simulink model "stabilizer_bar_repair"  (R2023a)
settings: Solver=ode4  StartTime=0  StopTime=40  FixedStep=Ts_plant  MaxStep=0.001  RelTol=1e-3
InitFcn:
  | run(fullfile(fileparts(get_param(bdroot,'FileName')),'a001_new_Design_LQR_Controller.m'));
values from neighbouring files (symbols this model uses):
  cycle_cfg = jsondecode(fileread(fullfile(repair_root,'repair_support','repair_cycle_bank.json')))    [a001_new_Design_LQR_Controller.m]
  entry_cfg = rmfield(entry_bank_source,{'labels','source_hashes','note','source_par_sha256'})    [a001_new_Design_LQR_Controller.m]
  path_geometry = repair_build_geometry(path_cfg)    [a001_new_Design_LQR_Controller.m]
  path_Q = diag([10,10,2])    [a001_new_Design_LQR_Controller.m]
  path_R = diag([100,100,10])    [a001_new_Design_LQR_Controller.m]
  repair_cfg = struct    [a001_new_Design_LQR_Controller.m]
  repair_simfile = 'C:\Users\Public\Documents\CarSim2020.0_Data\Extensions\Simulink\00carsim_workspace\009\stabilizer_bar\simfile.sim'    [a001_new_Design_LQR_Controller.m]
  stadium_cfg = jsondecode(fileread(fullfile(repair_root,'repair_support','repair_stadium_reference.json')))    [a001_new_Design_LQR_Controller.m]
  Ts = 0.01    [a001_new_Design_LQR_Controller.m]
  Ts_plant = 0.0005    [a001_new_Design_LQR_Controller.m]
undefined symbols (not defined in the file or in its folder): path_cfg
(part 1 of 2)
settings Model: Creator=28583  LastModifiedBy=28583

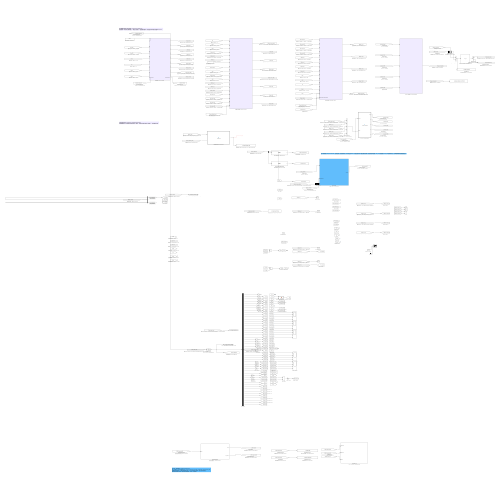
[thumbnail: Simulink's stored preview of the top-level diagram]
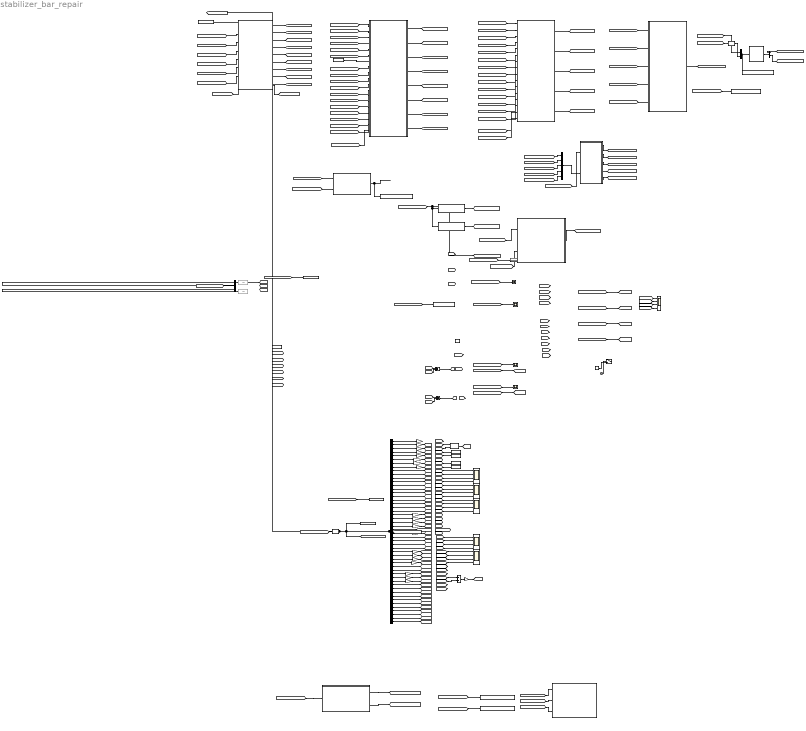
== system stabilizer_bar_repair ==
  note: 第四章路径跟踪与分阶段维修 / Chapter 4 Staged Repair
      | 路径跟踪 → 状态与力需求修正 → 轮速/力矩执行 → 直接前轮角接口。跨层信号均采用本层局部Goto/From。
  note: 诊断与实际状态 / Diagnostics and Measured States
      | 保留原始需求、修正残差和未滤波数据；无候选、轮荷失效或坐标失效立即停止，不开展增益扫描。
  note: 起漂与局部维持 / Entry & Local Hold：工程试验支路，路径反馈关闭。工作点来自当前CarSim；先建立后轴滑移，再建立横摆与负侧偏，最后按实测状态接管。drift_entry仅起漂维持；drift_cycle按实测状态门控，经卸载和解除转弯后接管普通直行。
  note: 第一阶段：固定软硬组合 / Fixed Active Roll Study
      | 唯一入口a001；asb_case选择baseline、front_soft_rear_hard、soft_soft、hard_hard、front_hard_rear_soft。
      | 原漂移控制与路线冻结，新增支路按0.0005s执行。CarSim内部384/384不动，输出比较不预设优劣。
      | 跨区信号均为本层local标签；新增支路不增加滤波、延迟或人为表端停止。
  ASBExportSplit : Demux  Outputs=[50 26]
      settings: AttributesFormatString=原50路与新增26路 / Split Export
  ASBImport12 : Mux  Inputs=2
      settings: AttributesFormatString=12路CarSim输入 / Import Twelve
  ASBImportOrder : Selector  InputPortWidth=4  IndexOptions=Index vector (dialog)  Indices=[1 3 2 4]  OutputSizes=1
      settings: AttributesFormatString=GUI轮序重排 / GUI Force Order
  ActiveRollMonitor : Subsystem
      settings: AttributesFormatString=主动稳定杆诊断面板 / Active Roll Monitor
  ActiveRollResearch : Subsystem
      settings: AttributesFormatString=理想主动稳定杆 / Ideal Active Roll
  ActualStateSample 车辆状态采样模块 : ZeroOrderHold  SampleTime=Ts
      settings: AttributesFormatString=|
      | ActualStateSample
      | 车辆状态采样模块 / ActualStateSample
  Add : Sum
      settings: AttributesFormatString=Add / Add
  Add1 : Sum
      settings: AttributesFormatString=Add1 / Add1
  Add2 : Sum
      settings: AttributesFormatString=Add2 / Add2
  CarSim S-Function : S-Function  Priority=1  FunctionName=vs_sf  Parameters=repair_simfile,2,0  SFunctionDeploymentMode=off  EnableBusSupport=off
      settings: AttributesFormatString=CarSim S-Function / CarSimSFunction
  CarSimInterface : Subsystem
      settings: AttributesFormatString=CarSim八路接口 / CarSimInterface
  Clock : Clock
      settings: AttributesFormatString=Clock / Clock
  Constant1 : Constant  Value=Ts
      settings: AttributesFormatString=Constant1 / Constant1
  Constant8 : Constant  Value=-7.37
      settings: AttributesFormatString=Constant8 / Constant8
  Demux : Demux  Outputs=50
      settings: AttributesFormatString=Demux / Demux
  Display : Display
      settings: AttributesFormatString=Display / Display
  EntryLocalMode : Subsystem
      settings: AttributesFormatString=起漂维持退出与直行 / Drift Cycle
  EntryModeSelector : MATLAB Function  TreatAsAtomicUnit=on
      settings: AttributesFormatString=运行模式选择 / Mode Selection
  Gain1 : Gain  Gain=1/3.6
      settings: AttributesFormatString=Gain1 / Gain1
  Gain{7,10..12,16,18..20} (8 alike) : Gain  Gain=pi/30
      Gain10 settings: AttributesFormatString=Gain10 / Gain10
      Gain11 settings: AttributesFormatString=Gain11 / Gain11
      Gain12 settings: AttributesFormatString=Gain12 / Gain12
      Gain16 settings: AttributesFormatString=Gain16 / Gain16
      Gain18 settings: AttributesFormatString=Gain18 / Gain18
      Gain19 settings: AttributesFormatString=Gain19 / Gain19
      Gain20 settings: AttributesFormatString=Gain20 / Gain20
      Gain7 settings: AttributesFormatString=Gain7 / Gain7
  Gain{4..6,9,13,21..22} (7 alike) : Gain  Gain=pi/180
      Gain13 settings: AttributesFormatString=Gain13 / Gain13
      Gain21 settings: AttributesFormatString=Gain21 / Gain21
      Gain22 settings: AttributesFormatString=Gain22 / Gain22
      Gain4 settings: AttributesFormatString=Gain4 / Gain4
      Gain5 settings: AttributesFormatString=Gain5 / Gain5
      Gain6 settings: AttributesFormatString=Gain6 / Gain6
      Gain9 settings: AttributesFormatString=Gain9 / Gain9
  Gain14 : Gain  Gain=1/3.6
      settings: AttributesFormatString=Gain14 / Gain14
  Gain15 : Gain  Gain=9.80665
      settings: AttributesFormatString=Gain15 / Gain15
  Gain2 : Gain  Gain=1/3.6
      settings: AttributesFormatString=Gain2 / Gain2
  Gain3 : Gain  Gain=9.80665
      settings: AttributesFormatString=Gain3 / Gain3
  Gain8 : Gain  Gain=1/2
      settings: AttributesFormatString=Gain8 / Gain8
  LegacyCommand5 : Mux  Inputs=5
      settings: AttributesFormatString=原模式指令 / Legacy Commands
  LogASBDiagnostics : ToWorkspace  VariableName=asb_diag  SaveFormat=Structure With Time  SampleTime=-1
      settings: AttributesFormatString=记录力矩功率残差 / Log ASB Diagnostics
  LogASBImport : ToWorkspace  VariableName=asb_import12  SaveFormat=Structure With Time  SampleTime=-1
      settings: AttributesFormatString=记录12路实际输入 / Log Full Import
  LogASBSuspension : ToWorkspace  VariableName=asb_suspension  SaveFormat=Structure With Time  SampleTime=-1
      settings: AttributesFormatString=记录悬架26路 / Log Suspension
  Log_repair_actuator_command : ToWorkspace  VariableName=repair_actuator_command  SaveFormat=Timeseries  SampleTime=-1
      settings: AttributesFormatString=Log_repair_actuator_command / Log_repair_actuator_command
  Log_repair_path_diag : ToWorkspace  VariableName=repair_path_diag  SaveFormat=Timeseries  SampleTime=-1
      settings: AttributesFormatString=原始路径日志 / Log_repair_path_diag
  Log_repair_plant_raw : ToWorkspace  VariableName=repair_plant_raw  SaveFormat=Timeseries  SampleTime=-1
      settings: AttributesFormatString=Log_repair_plant_raw / Log_repair_plant_raw
  Log_repair_plant_sampled : ToWorkspace  VariableName=repair_plant_sampled  SaveFormat=Timeseries  SampleTime=-1
      settings: AttributesFormatString=Log_repair_plant_sampled / Log_repair_plant_sampled
  Log_repair_reference_log : ToWorkspace  VariableName=repair_reference_log  SaveFormat=Timeseries  SampleTime=-1
      settings: AttributesFormatString=Log_repair_reference_log / Log_repair_reference_log
  Log_repair_stage_stop : ToWorkspace  VariableName=repair_stage_stop  SaveFormat=Timeseries  SampleTime=-1
      settings: AttributesFormatString=原始记录 repair_stage_stop / Log_repair_stage_stop
  MATLAB Function : MATLAB Function  TreatAsAtomicUnit=on
      settings: AttributesFormatString=MATLAB Function / MATLABFunction
  MeasuredFourWheelLoads : Selector  InputPortWidth=50  IndexOptions=Index vector (dialog)  Indices=17:20  OutputSizes=1
      settings: AttributesFormatString=四轮实际轮荷 / Measured Fz [N]
  PathClock : DigitalClock  SampleTime=Ts
      settings: AttributesFormatString=控制采样时刻 / PathClock
  ReferenceSignals : Demux  Outputs=3
      settings: AttributesFormatString=ReferenceSignals / ReferenceSignals
  RepairClock : DigitalClock  SampleTime=Ts
      settings: AttributesFormatString=控制采样时刻 / RepairClock
  RepairTs : Constant  Value=Ts
      settings: AttributesFormatString=控制周期参数 / RepairTs
  Scope{,2,7,9,13,21} (6 alike) : Scope  NumInputPorts=4
      Scope settings: AttributesFormatString=Scope / Scope
      Scope13 settings: AttributesFormatString=Scope13 / Scope13
      Scope2 settings: AttributesFormatString=Scope2 / Scope2
      Scope21 settings: AttributesFormatString=Scope21 / Scope21
      Scope7 settings: AttributesFormatString=Scope7 / Scope7
      Scope9 settings: AttributesFormatString=Scope9 / Scope9
  Scope{14..17} (4 alike) : Scope
      Scope14 settings: AttributesFormatString=Scope14 / Scope14
      Scope15 settings: AttributesFormatString=Scope15 / Scope15
      Scope16 settings: AttributesFormatString=Scope16 / Scope16
      Scope17 settings: AttributesFormatString=Scope17 / Scope17
  StageStop : MATLAB Function  Description=|  TreatAsAtomicUnit=on
      | 停止逻辑已移除 / Stop logic removed
      | 阶段状态仅作为日志信号，CarSim/求解器按自身行为终止。
      settings: AttributesFormatString=分阶段停止条件 / StageStop
  Switch : Switch  Criteria=u2 > Threshold  Threshold=0.5  SaturateOnIntegerOverflow=off  InputSameDT=off
      settings: AttributesFormatString=Switch / Switch
  To Workspace1 : ToWorkspace  VariableName=beta_out1  SaveFormat=Timeseries  SampleTime=-1
      settings: AttributesFormatString=To Workspace1 / ToWorkspace1
  To Workspace2 : ToWorkspace  VariableName=AVz_out1  SaveFormat=Timeseries  SampleTime=-1
      settings: AttributesFormatString=To Workspace2 / ToWorkspace2
  To Workspace3 : ToWorkspace  VariableName=Roll_out1  SaveFormat=Timeseries  SampleTime=-1
      settings: AttributesFormatString=To Workspace3 / ToWorkspace3
  To Workspace4 : ToWorkspace  VariableName=Ay_out1  SaveFormat=Timeseries  SampleTime=-1
      settings: AttributesFormatString=To Workspace4 / ToWorkspace4
  Transfer Fcn1 : TransferFcn  Commented=through  Denominator=[1 1]
  Transfer Fcn2 : TransferFcn  Commented=through  Denominator=[1 1]
  WheelContactSelector : Selector  InputPortWidth=50  IndexOptions=Index vector (dialog)  Indices=[9 10 11 12 17 18 19 20]  OutputSizes=1
      settings: AttributesFormatString=轮胎负载与轮荷 / Wheel Contact
  执行器调节层 : Subsystem  Description=|
      | 执行命令直通 / Unbounded Commands to CarSim
      | 关闭外加转角、角速度、轮速变化及轮端力矩限幅。
      | 非有限值和CarSim求解器错误由CarSim/求解器本身反映。
      settings: AttributesFormatString=执行器调节 / Actuator Control
  路径跟踪层 : Subsystem  Description=|
      | 普通工况mode=6：直线→平滑左转→直线。
      | 漂移权重与侧偏参考始终为零。
      | 主链仍为参考对齐→位姿误差→LQR→期望状态；保留原控制增益。
      settings: AttributesFormatString=路径跟踪 / Path Tracking
  车辆运动控制层 : Subsystem  Description=|
      | 状态参考直通 / Unconstrained Reference Pass-through
      | 完整LQR状态命令不再经过33点可行域搜索、5%轴力残差门槛或摩擦圆投影。
      | CarSim实际Fx/Fy/Fz、滑移和车辆状态用于判断命令后果。
      settings: AttributesFormatString=车辆运动控制 / Motion Control
  wires:
  ActualStateSample 车辆状态采样模块/1 -> Demux/1, [Repair_sampled_plant], [Repair_HeldPlant], Log_repair_plant_sampled/1, [Stadium_Measured]
  Add/1 -> [Fzf]
  Add1/1 -> [Fzr]
  Add2/1 -> Gain8/1
  [Ay] -> To Workspace4/1
  CarSimInterface/1(CarSimInputs) -> [Repair_commands]
  Clock/1 -> Switch/2
  Constant8/1 -> Switch/3
  Demux/1 -> Gain14/1
  Demux/2 -> Gain1/1
  Demux/3 -> Gain2/1
  Demux/4 -> Gain4/1
  Demux/5 -> Gain5/1
  Demux/6 -> Gain3/1
  Demux/7 -> Gain15/1
  Demux/8 -> Gain6/1
  Demux/9 -> [Fx_L1]
  Demux/10 -> [Fx_R1]
  Demux/11 -> [Fx_L2]
  Demux/12 -> [Fx_R2]
  Demux/13 -> [Fy_L1]
  Demux/14 -> [Fy_R1]
  Demux/15 -> [Fy_L2]
  Demux/16 -> [Fy_R2]
  Demux/17 -> [Fz_L1]
  Demux/18 -> [Fz_R1]
  Demux/19 -> [Fz_L2]
  Demux/20 -> [Fz_R2]
  Demux/21 -> Gain16/1
  Demux/22 -> Gain18/1
  Demux/23 -> Gain19/1
  Demux/24 -> Gain20/1
  Demux/25 -> [Steer_wheel_angular_rate]
  Demux/26 -> Gain9/1
  Demux/27 -> [Kappa_L1]
  Demux/28 -> [Kappa_R1]
  Demux/29 -> [Kappa_L2]
  Demux/30 -> [Kappa_R2]
  Demux/31 -> Gain7/1
  Demux/32 -> Gain10/1
  Demux/33 -> Gain11/1
  Demux/34 -> Gain12/1
  Demux/35 -> [Xcg_TM]
  Demux/36 -> [Ycg_TM]
  Demux/37 -> Gain13/1
  Demux/38 -> Gain21/1
  Demux/39 -> Gain22/1
  Demux/40 -> [Xo]
  Demux/41 -> [Yo]
  Demux/42 -> [My_Dr_L1]
  Demux/43 -> [My_Dr_R1]
  Demux/44 -> [My_Dr_L2]
  Demux/45 -> [My_Dr_R2]
  Demux/46 -> [Alpha_L1]
  Demux/47 -> [Alpha_R1]
  Demux/48 -> [Alpha_L2]
  Demux/49 -> [Alpha_R2]
  Demux/50 -> [Steer_SW]
  [wheel_steer_L1] -> Add2/1
  [Fz_L1] -> Add/1
  [Fz_R1] -> Add/2
  [Fz_L2] -> Add1/1
  [Fz_R2] -> Add1/2
  [wheel_steer_R1] -> Add2/2
  [IMP_MY_OUT_L1] -> Scope7/1
  [IMP_MY_OUT_R1] -> Scope7/2
  [AVy_wheel_L1] -> Scope21/1
  [IMP_MY_OUT_L2] -> Scope7/3
  [IMP_MY_OUT_R2] -> Scope7/4
  [AVy_wheel_R1] -> Scope21/2
  [AVy_wheel_L2] -> Scope21/3
  [AVy_wheel_R2] -> Scope21/4
  [Fx_L1] -> Scope9/1
  [Fx_L2] -> Scope9/3
  [Fx_R1] -> Scope9/2
  [Fx_R2] -> Scope9/4
  [Fy_L1] -> Scope2/1
  [Fy_L2] -> Scope2/3
  [Fy_R1] -> Scope2/2
  [Fy_R2] -> Scope2/4
  [Fz_L1] -> Scope/1
  [Fz_L2] -> Scope/3
  [Fz_R1] -> Scope/2
  [Fz_R2] -> Scope/4
  Gain1/1 -> [Vx]
  Gain10/1 -> [AVy_wheel_R1]
  Gain11/1 -> [AVy_wheel_L2]
  Gain12/1 -> [AVy_wheel_R2]
  Gain13/1 -> [Yaw]
  Gain15/1 -> [Ay]
  Gain16/1 -> [AVy_L1]
  Gain18/1 -> [AVy_R1]
  Gain19/1 -> [AVy_L2]
  Gain2/1 -> [Vy]
  Gain20/1 -> [AVy_R2]
  Gain21/1 -> [wheel_steer_L1]
  Gain22/1 -> [wheel_steer_R1]
  Gain3/1 -> [Ax]
  Gain4/1 -> [beta]
  Gain5/1 -> [AVz]
  Gain6/1 -> [Roll]
  Gain7/1 -> [AVy_wheel_L1]
  Gain8/1 -> [delta_acutal_F]
  Gain9/1 -> [AVx]
  [Kappa_L1] -> Scope13/1
  [Kappa_L2] -> Scope13/3
  [Kappa_R1] -> Scope13/2
  [Kappa_R2] -> Scope13/4
  MATLAB Function/1(V) -> [V]
  [Repair_plant_raw] -> ActualStateSample 车辆状态采样模块/1
  [Repair_inverse_status] -> Display/1
  [Repair_T_FL] -> [IMP_MY_OUT_L1]
  [Repair_T_FR] -> [IMP_MY_OUT_R1]
  [Repair_T_RL] -> [IMP_MY_OUT_L2]
  [Repair_Fxf] -> [Fxf_desire]
  [Repair_Fxr] -> [Fxr_desire]
  [Repair_T_RR] -> [IMP_MY_OUT_R2]
  [Repair_plant_raw] -> Log_repair_plant_raw/1
  [Repair_path_diag] -> Log_repair_path_diag/1
  [Repair_nominal] -> Log_repair_reference_log/1
  [Repair_nominal] -> ReferenceSignals/1
  [Repair_commands] -> Log_repair_actuator_command/1
  [Repair_sampled_plant] -> StageStop/2(plant)
  [Repair_wf] -> Scope14/1
  [Repair_wr] -> Scope15/1
  [Repair_Fxf] -> Scope16/1
  [Repair_Fxr] -> Scope17/1
  [Repair_valid] -> StageStop/1(valid)
  [Fzr] -> 执行器调节层/10(后轴垂向力)
  [Repair_blend] -> 车辆运动控制层/10(漂移模式1_0drift_mode)
  [Fzf] -> 车辆运动控制层/11(前轴垂向载荷Fzf)
  [V] -> 执行器调节层/11(V)
  [Repair_ey] -> 车辆运动控制层/12(PathLateralError)
  [beta] -> 执行器调节层/12(beta)
  [AVz] -> 执行器调节层/13(r)
  [Repair_chi] -> 车辆运动控制层/13(PathCourseError)
  [Repair_alpha] -> 执行器调节层/14(期望前轮侧偏角alpha_f_d)
  [Repair_kappa] -> 车辆运动控制层/14(PathCurvature)
  [AVy_wheel_L1] -> 车辆运动控制层/15(WheelSpeed1)
  [AVy_wheel_R1] -> 车辆运动控制层/16(WheelSpeed2)
  [AVy_wheel_L2] -> 车辆运动控制层/17(WheelSpeed3)
  [AVy_wheel_R2] -> 车辆运动控制层/18(WheelSpeed4)
  [AVy_wheel_L1] -> 执行器调节层/1(左前轮实际轮速)
  [V] -> 车辆运动控制层/1(实际速度V)
  [AVy_wheel_R1] -> 执行器调节层/2(右前轮实际轮速)
  [Xcg_TM] -> 路径跟踪层/2(Xcg)
  [beta] -> 车辆运动控制层/2(质心侧偏角beta)
  [AVy_wheel_L2] -> 执行器调节层/3(左后轮实际轮速)
  [AVz] -> 车辆运动控制层/3(横摆角速度r)
  [Ycg_TM] -> 路径跟踪层/3(Ycg)
  [AVy_wheel_R2] -> 执行器调节层/4(右后轮实际轮速)
  [Repair_Vxd] -> 车辆运动控制层/4(路径跟踪层输出的期望纵向速度Vxd)
  [Yaw] -> 路径跟踪层/4(Yaw)
  [Repair_Vyd] -> 车辆运动控制层/5(路径跟踪层输出的期望侧向速度Vyd)
  [Repair_wf] -> 执行器调节层/5(前轴期望轴轮速)
  [V] -> 路径跟踪层/5(Speed)
  [Repair_rd] -> 车辆运动控制层/6(路径跟踪层输出的期望横摆角速度rd_in)
  [Repair_wr] -> 执行器调节层/6(后轴期望轴轮速)
  [beta] -> 路径跟踪层/6(Beta)
  [AVz] -> 路径跟踪层/7(YawRate)
  [Repair_Fxf] -> 执行器调节层/7(前轴期望纵向力)
  [Repair_Fxr] -> 执行器调节层/8(后轴期望纵向力)
  [delta_acutal_F] -> 车辆运动控制层/8(前轮转角delta_f)
  [Fzf] -> 执行器调节层/9(前轴垂向力)
  [Fzr] -> 车辆运动控制层/9(后轴垂向载荷Fzr)
  ReferenceSignals/1 -> [V_refer]
  ReferenceSignals/2 -> Transfer Fcn1/1
  ReferenceSignals/3 -> Transfer Fcn2/1
  RepairClock/1 -> 路径跟踪层/1(Time)
  RepairTs/1 -> 车辆运动控制层/7(采样时间)
  [Roll] -> To Workspace3/1
  StageStop/1(stop) -> Log_repair_stage_stop/1
  [Vx] -> MATLAB Function/1(Vx)
  [Vy] -> MATLAB Function/2(Vy)
  [beta] -> To Workspace1/1
  [AVz] -> To Workspace2/1
  执行器调节层/1(左前轮驱动力矩) -> [Repair_T_FL]
  执行器调节层/2(右前轮驱动力矩) -> [Repair_T_FR]
  执行器调节层/3(左后轮驱动力矩) -> [Repair_T_RL]
  执行器调节层/4(右后轮驱动力矩) -> [Repair_T_RR]
  执行器调节层/5(FrontAngleCommand) -> [Repair_delta_target]
  路径跟踪层/1(Vxd) -> [Repair_Vxd]
  路径跟踪层/2(Vyd) -> [Repair_Vyd]
  路径跟踪层/3(rd) -> [Repair_rd]
  路径跟踪层/4(LateralError) -> [Repair_ey]
  路径跟踪层/5(CourseError) -> [Repair_chi]
  路径跟踪层/6(ProjectedCurvature) -> [Repair_kappa]
  路径跟踪层/7(DriftBlend) -> [Repair_blend]
  路径跟踪层/8(PathDiagnostics) -> [Repair_path_diag]
  路径跟踪层/9(NominalStates) -> [Repair_nominal]
  车辆运动控制层/1(漂移状态status) -> [Repair_inverse_status]
  车辆运动控制层/2(期望前轴轮速1) -> [Repair_wf]
  车辆运动控制层/3(期望后轴轮速1) -> [Repair_wr]
  车辆运动控制层/4(期望前轮侧偏角2) -> [Repair_alpha]
  车辆运动控制层/5(轮胎反演状态1) -> [Repair_force_valid]
  车辆运动控制层/6(期望前轮纵向力Fxf) -> [Repair_Fxf]
  车辆运动控制层/7(期望后轮纵向力Fxr) -> [Repair_Fxr]
  车辆运动控制层/8(Feasible) -> [Repair_valid]
  WheelContactSelector/1 -> [Repair_WheelContact]
  [Repair_WheelContact] -> 车辆运动控制层/19(MeasuredWheelContact)
  [Repair_WheelContact] -> 执行器调节层/15(MeasuredWheelContact)
  [Repair_HeldPlant] -> WheelContactSelector/1, MeasuredFourWheelLoads/1, [entry_plant50]
  MeasuredFourWheelLoads/1 -> [measured_Fz4]
  [measured_Fz4] -> 执行器调节层/16(MeasuredFourWheelLoads)
  [Repair_delta_target] -> LegacyCommand5/1
  [Repair_T_FL] -> LegacyCommand5/2
  [Repair_T_FR] -> LegacyCommand5/3
  [Repair_T_RL] -> LegacyCommand5/4
  [Repair_T_RR] -> LegacyCommand5/5
  [entry_command5] -> EntryModeSelector/1(newcmd)
  LegacyCommand5/1 -> EntryModeSelector/2(oldcmd)
  EntryModeSelector/1(angle) -> [selected_Angle]
  [selected_Angle] -> CarSimInterface/1(Input1)
  EntryModeSelector/2(tfl) -> [selected_TFL]
  [selected_TFL] -> CarSimInterface/2(Input2)
  EntryModeSelector/3(tfr) -> [selected_TFR]
  [selected_TFR] -> CarSimInterface/3(Input3)
  EntryModeSelector/4(trl) -> [selected_TRL]
  [selected_TRL] -> CarSimInterface/4(Input4)
  EntryModeSelector/5(trr) -> [selected_TRR]
  [selected_TRR] -> CarSimInterface/5(Input5)
  [entry_plant50] -> EntryLocalMode/1(y)
  EntryLocalMode/1(command) -> [entry_command5]
  [Stadium_Measured] -> 路径跟踪层/8(StadiumRaw)
  路径跟踪层/10(StadiumPacket) -> [Stadium_Packet]
  [Stadium_Packet] -> EntryLocalMode/2(StadiumPacket)
  [Repair_commands] -> ASBImport12/1
  [ASB_Force4] -> ASBImportOrder/1
  ASBImportOrder/1 -> ASBImport12/2
  ASBImport12/1 -> CarSim S-Function/1, LogASBImport/1
  CarSim S-Function/1 -> ASBExportSplit/1
  ASBExportSplit/1 -> [Repair_plant_raw]
  ASBExportSplit/2 -> [ASB_Suspension26]
  [ASB_Suspension26] -> ActiveRollResearch/1(Raw)
  ActiveRollResearch/1(Forces) -> [ASB_Force4]
  ActiveRollResearch/2(Diagnostics) -> [ASB_Diagnostics44]
  [ASB_Diagnostics44] -> LogASBDiagnostics/1
  [ASB_Suspension26] -> LogASBSuspension/1
  [ASB_Diagnostics44] -> ActiveRollMonitor/1(Diagnostics)
  [ASB_Suspension26] -> ActiveRollMonitor/2(Suspension)
  [Repair_plant_raw] -> ActiveRollMonitor/3(Vehicle)

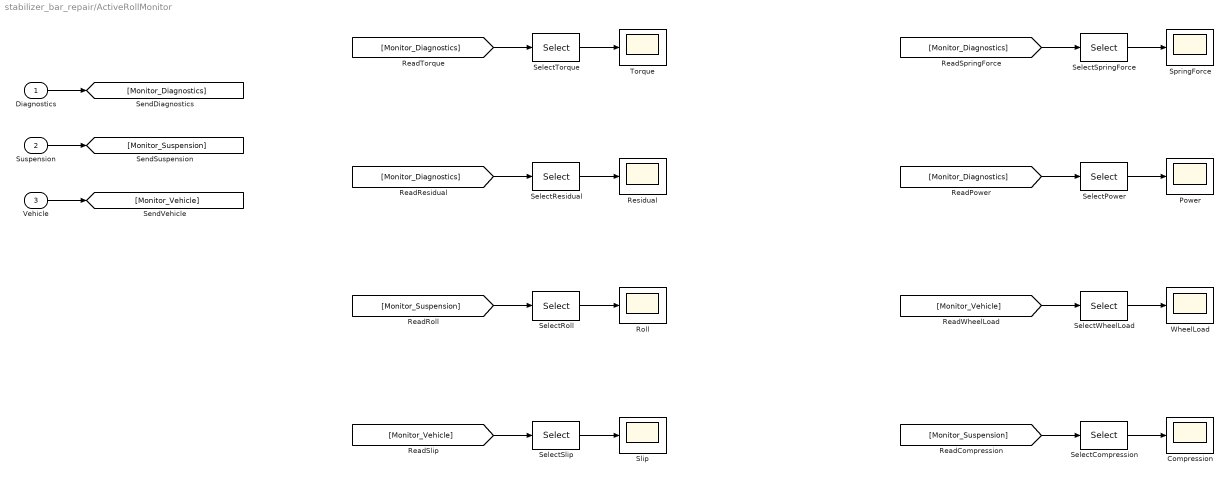
== system stabilizer_bar_repair/ActiveRollMonitor ==
  Diagnostics : Inport  PortDimensions=44
      settings: AttributesFormatString=44项物理诊断 / Diagnostics
  Suspension : Inport  Port=2  PortDimensions=26
      settings: AttributesFormatString=26路悬架测量 / Suspension
  Vehicle : Inport  Port=3  PortDimensions=50
      settings: AttributesFormatString=50路车辆测量 / Vehicle
  Compression : Scope
      settings: AttributesFormatString=|
      | 四轮弹簧压缩 mm
      | Spring Compression
  Power : Scope
      settings: AttributesFormatString=|
      | 两口径机械功率与差值 W
      | Power
  Residual : Scope
      settings: AttributesFormatString=|
      | 力矩残差Nm与合力N
      | Residual
  Roll : Scope
      settings: AttributesFormatString=|
      | 相对侧倾deg及速度deg每秒
      | Relative Roll
  SelectCompression : Selector  InputPortWidth=26  IndexOptions=Index vector (dialog)  Indices=[17:20]  OutputSizes=1
      settings: AttributesFormatString=选取 / Select
  SelectPower : Selector  InputPortWidth=44  IndexOptions=Index vector (dialog)  Indices=[29:34]  OutputSizes=1
      settings: AttributesFormatString=选取 / Select
  SelectResidual : Selector  InputPortWidth=44  IndexOptions=Index vector (dialog)  Indices=[11 12 27 28]  OutputSizes=1
      settings: AttributesFormatString=选取 / Select
  SelectRoll : Selector  InputPortWidth=26  IndexOptions=Index vector (dialog)  Indices=[1:4]  OutputSizes=1
      settings: AttributesFormatString=选取 / Select
  SelectSlip : Selector  InputPortWidth=50  IndexOptions=Index vector (dialog)  Indices=[27:30]  OutputSizes=1
      settings: AttributesFormatString=选取 / Select
  SelectSpringForce : Selector  InputPortWidth=44  IndexOptions=Index vector (dialog)  Indices=[19:26]  OutputSizes=1
      settings: AttributesFormatString=选取 / Select
  SelectTorque : Selector  InputPortWidth=44  IndexOptions=Index vector (dialog)  Indices=[7:10]  OutputSizes=1
      settings: AttributesFormatString=选取 / Select
  SelectWheelLoad : Selector  InputPortWidth=50  IndexOptions=Index vector (dialog)  Indices=[17:20]  OutputSizes=1
      settings: AttributesFormatString=选取 / Select
  Slip : Scope
      settings: AttributesFormatString=|
      | 四轮纵滑比
      | Longitudinal Slip
  SpringForce : Scope
      settings: AttributesFormatString=|
      | 四轮输入与实际弹簧力 N
      | Spring Force
  Torque : Scope
      settings: AttributesFormatString=|
      | 前后目标与实际力矩 Nm
      | Torque
  WheelLoad : Scope
      settings: AttributesFormatString=|
      | 四轮法向载荷 N
      | Wheel Load
  wires:
  Diagnostics/1 -> [Monitor_Diagnostics]
  Suspension/1 -> [Monitor_Suspension]
  Vehicle/1 -> [Monitor_Vehicle]
  [Monitor_Diagnostics] -> SelectTorque/1
  SelectTorque/1 -> Torque/1
  [Monitor_Diagnostics] -> SelectSpringForce/1
  SelectSpringForce/1 -> SpringForce/1
  [Monitor_Diagnostics] -> SelectResidual/1
  SelectResidual/1 -> Residual/1
  [Monitor_Diagnostics] -> SelectPower/1
  SelectPower/1 -> Power/1
  [Monitor_Suspension] -> SelectRoll/1
  SelectRoll/1 -> Roll/1
  [Monitor_Vehicle] -> SelectWheelLoad/1
  SelectWheelLoad/1 -> WheelLoad/1
  [Monitor_Vehicle] -> SelectSlip/1
  SelectSlip/1 -> Slip/1
  [Monitor_Suspension] -> SelectCompression/1
  SelectCompression/1 -> Compression/1

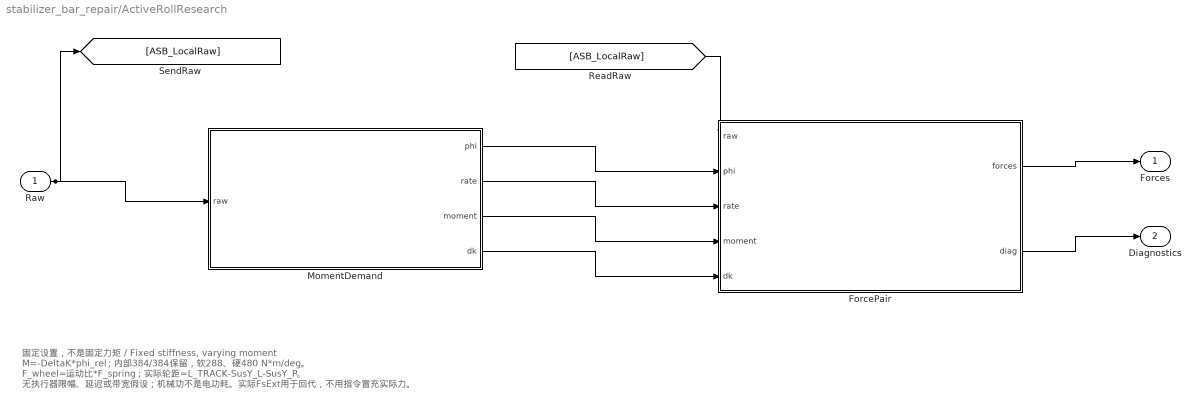
== system stabilizer_bar_repair/ActiveRollResearch ==
  note: 固定设置，不是固定力矩 / Fixed stiffness, varying moment
      | M=-DeltaK*phi_rel；内部384/384保留，软288、硬480 N*m/deg。
      | F_wheel=运动比*F_spring；实际轮距=L_TRACK-SusY_L-SusY_R。
      | 无执行器限幅、延迟或带宽假设；机械功不是电功耗。实际FsExt用于回代，不用指令冒充实际力。
  Raw : Inport  PortDimensions=26
      settings: AttributesFormatString=悬架26路 / Suspension Raw
  ForcePair : MATLAB Function  TreatAsAtomicUnit=on
      settings: AttributesFormatString=运动比力偶与回代 / Force Pair
  MomentDemand : MATLAB Function  TreatAsAtomicUnit=on
      settings: AttributesFormatString=固定刚度与恢复力矩 / Moment Demand
  Forces : Outport
      settings: AttributesFormatString=弹簧力FL FR RL RR / Spring Forces
  Diagnostics : Outport  Port=2
      settings: AttributesFormatString=44项物理诊断 / Diagnostics
  wires:
  Raw/1 -> MomentDemand/1(raw), [ASB_LocalRaw]
  [ASB_LocalRaw] -> ForcePair/1(raw)
  MomentDemand/1(phi) -> ForcePair/2(phi)
  MomentDemand/2(rate) -> ForcePair/3(rate)
  MomentDemand/3(moment) -> ForcePair/4(moment)
  MomentDemand/4(dk) -> ForcePair/5(dk)
  ForcePair/1(forces) -> Forces/1
  ForcePair/2(diag) -> Diagnostics/1

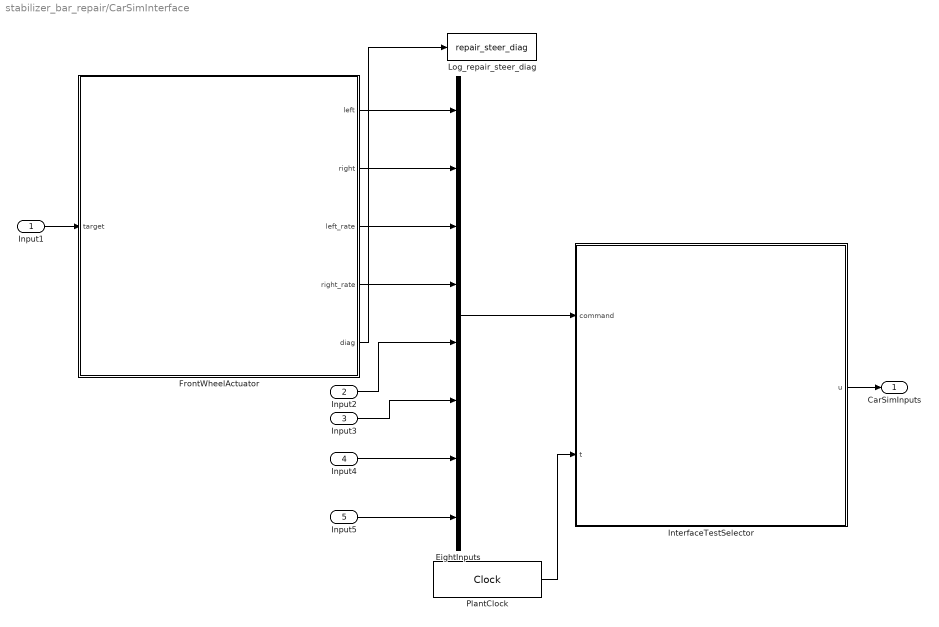
== system stabilizer_bar_repair/CarSimInterface ==
  Input1 : Inport
      settings: AttributesFormatString=Repair_delta_target / Input1
  Input2 : Inport  Port=2
      settings: AttributesFormatString=Repair_T_FL / Input2
  Input3 : Inport  Port=3
      settings: AttributesFormatString=Repair_T_FR / Input3
  Input4 : Inport  Port=4
      settings: AttributesFormatString=Repair_T_RL / Input4
  Input5 : Inport  Port=5
      settings: AttributesFormatString=Repair_T_RR / Input5
  EightInputs : Mux  Inputs=8
      settings: AttributesFormatString=CarSim输入顺序 / EightInputs
  FrontWheelActuator : MATLAB Function  TreatAsAtomicUnit=on
      settings: AttributesFormatString=前轮角与角速度 / FrontWheelActuator
  InterfaceTestSelector : MATLAB Function  TreatAsAtomicUnit=on
      settings: AttributesFormatString=显式接口短测选择 / InterfaceTestSelector
  Log_repair_steer_diag : ToWorkspace  VariableName=repair_steer_diag  SaveFormat=Timeseries  SampleTime=-1
      settings: AttributesFormatString=原始记录 repair_steer_diag / Log_repair_steer_diag
  PlantClock : DigitalClock  SampleTime=Ts_plant
      settings: AttributesFormatString=交换时刻 / PlantClock
  CarSimInputs : Outport
      settings: AttributesFormatString=八路导入向量 / CarSimInputs
  wires:
  Input3/1 -> EightInputs/6
  EightInputs/1 -> InterfaceTestSelector/1(command)
  Input2/1 -> EightInputs/5
  InterfaceTestSelector/1(u) -> CarSimInputs/1
  Input1/1 -> FrontWheelActuator/1(target)
  FrontWheelActuator/5(diag) -> Log_repair_steer_diag/1
  FrontWheelActuator/1(left) -> EightInputs/1
  FrontWheelActuator/2(right) -> EightInputs/2
  FrontWheelActuator/3(left_rate) -> EightInputs/3
  FrontWheelActuator/4(right_rate) -> EightInputs/4
  PlantClock/1 -> InterfaceTestSelector/2(t)
  Input4/1 -> EightInputs/7
  Input5/1 -> EightInputs/8

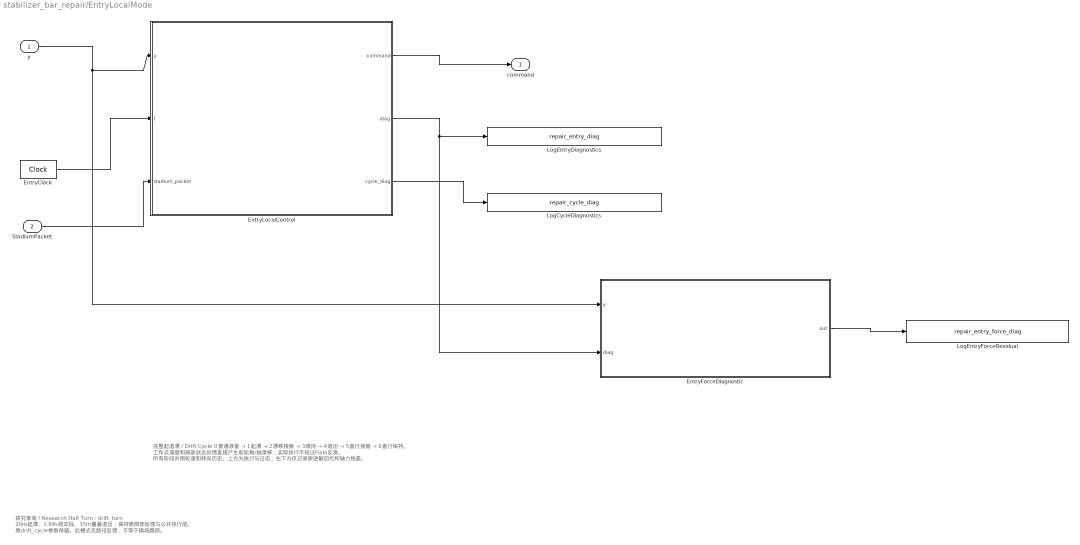
== system stabilizer_bar_repair/EntryLocalMode ==
  note: 完整起退漂 / Drift Cycle
      | 0普通准备 → 1起漂 → 2漂移接管 → 3维持 → 4退出 → 5直行接管 → 6直行保持。
      | 工作点调度和局部状态反馈直接产生前轮角/轴滑移；实际执行不经过Fiala反演。
      | 所有阶段共用轮速和转向历史。上方为执行与日志；右下方仅记录原逆解回代和轴力残差。
  note: 研究单弯 / Research Half Turn：drift_turn
      | 20m起漂、1.84s稳定段、35m重叠退出；保持原局部反馈与公共执行层。
      | 原drift_cycle参数保留。此模式无路径反馈，不等于操场跟踪。
  y : Inport
      settings: AttributesFormatString=实测状态 / Measured Plant
  StadiumPacket : Inport  Port=2
      settings: AttributesFormatString=操场执行参考 / Stadium Packet
  EntryClock : DigitalClock  SampleTime=Ts
      settings: AttributesFormatString=控制时钟 / Control Clock
  EntryForceDiagnostic : MATLAB Function  TreatAsAtomicUnit=on
      settings: AttributesFormatString=原逆解回代与力残差 / Inverse & Force Residual
  EntryLocalControl : MATLAB Function  TreatAsAtomicUnit=on
      settings: AttributesFormatString=五项状态反馈与执行 / Five-State Feedback and Execution
  LogCycleDiagnostics : ToWorkspace  VariableName=repair_cycle_diag  SaveFormat=Structure With Time  SampleTime=-1
      settings: AttributesFormatString=退出与直行接管记录 / Cycle Diagnostics
  LogEntryDiagnostics : ToWorkspace  VariableName=repair_entry_diag  SaveFormat=Structure With Time  SampleTime=-1
      settings: AttributesFormatString=起漂与接管记录 / Entry Diagnostics
  LogEntryForceResidual : ToWorkspace  VariableName=repair_entry_force_diag  SaveFormat=Structure With Time  SampleTime=-1
      settings: AttributesFormatString=轴力与回代记录 / Force Residual Log
  command : Outport
      settings: AttributesFormatString=前轮角与轮矩 / Actuator Command
  wires:
  y/1 -> EntryLocalControl/1(y), EntryForceDiagnostic/1(y)
  EntryClock/1 -> EntryLocalControl/2(t)
  EntryLocalControl/1(command) -> command/1
  EntryLocalControl/2(diag) -> LogEntryDiagnostics/1, EntryForceDiagnostic/2(diag)
  EntryLocalControl/3(cycle_diag) -> LogCycleDiagnostics/1
  EntryForceDiagnostic/1(out) -> LogEntryForceResidual/1
  StadiumPacket/1 -> EntryLocalControl/3(stadium_packet)

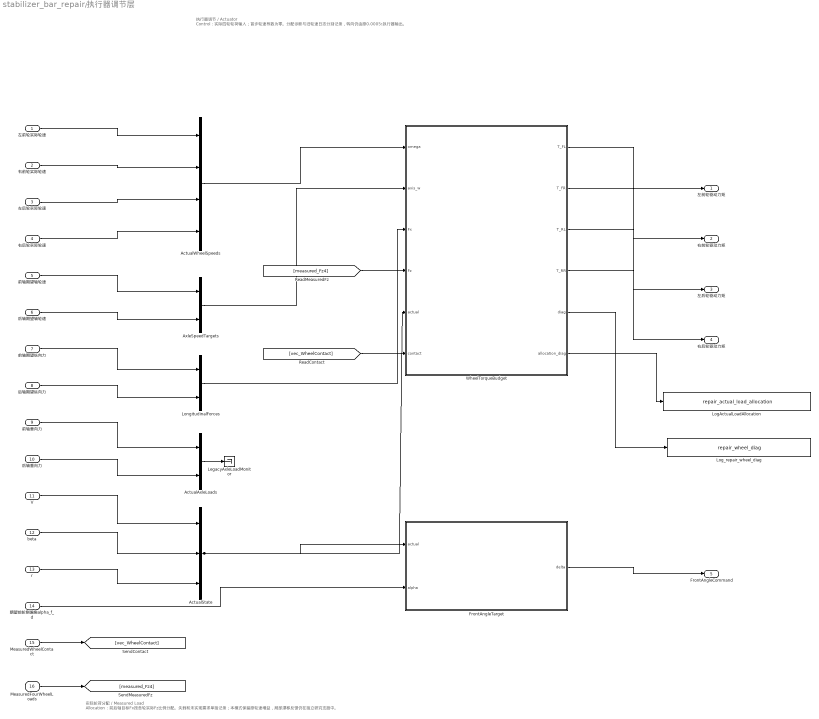
== system stabilizer_bar_repair/执行器调节层 ==
  note: 执行器调节 / Actuator Control：实际四轮轮荷输入；首步轮速导数为零。分配诊断与旧轮速日志分别记录，转向仍由原0.0005s执行器输出。
  note: 实际轮荷分配 / Measured Load Allocation：前后轴目标Fx按各轮实际Fz比例分配。失载和未实现需求单独记录；本模式保留原轮速增益，局部漂移反馈仍在独立研究支路中。
  左前轮实际轮速 : Inport
      settings: AttributesFormatString=左前实际轮速 / omega_FL
  右前轮实际轮速 : Inport  Port=2
      settings: AttributesFormatString=右前实际轮速 / omega_FR
  左后轮实际轮速 : Inport  Port=3
      settings: AttributesFormatString=左后实际轮速 / omega_RL
  右后轮实际轮速 : Inport  Port=4
      settings: AttributesFormatString=右后实际轮速 / omega_RR
  前轴期望轴轮速 : Inport  Port=5
      settings: AttributesFormatString=前轴候选轮速 / omega_f
  后轴期望轴轮速 : Inport  Port=6
      settings: AttributesFormatString=后轴候选轮速 / omega_r
  前轴期望纵向力 : Inport  Port=7
      settings: AttributesFormatString=前轴目标纵向力 / Fxf
  后轴期望纵向力 : Inport  Port=8
      settings: AttributesFormatString=后轴目标纵向力 / Fxr
  前轴垂向力 : Inport  Port=9
      settings: AttributesFormatString=前轴实际载荷 / Fzf
  后轴垂向力 : Inport  Port=10
      settings: AttributesFormatString=后轴实际载荷 / Fzr
  V : Inport  Port=11
      settings: AttributesFormatString=实际总速度 / V
  beta : Inport  Port=12
      settings: AttributesFormatString=实际侧偏角 / beta
  r : Inport  Port=13
      settings: AttributesFormatString=实际横摆角速度 / r
  期望前轮侧偏角alpha_f_d : Inport  Port=14
      settings: AttributesFormatString=前轴目标侧偏角 / alpha_f
  MeasuredWheelContact : Inport  Port=15
      settings: AttributesFormatString=实测轮胎负载 / Contact
  MeasuredFourWheelLoads : Inport  Port=16
      settings: AttributesFormatString=四轮实际轮荷 / Measured Fz [N]
  ActualAxleLoads : Mux  Inputs=2
      settings: AttributesFormatString=实际前后轴轮荷 / ActualAxleLoads
  ActualState : Mux  Inputs=3
      settings: AttributesFormatString=实际V beta r / ActualState
  ActualWheelSpeeds : Mux
      settings: AttributesFormatString=四轮实际轮速 / ActualWheelSpeeds
  AxleSpeedTargets : Mux  Inputs=2
      settings: AttributesFormatString=前后轴候选轮速 / AxleSpeedTargets
  FrontAngleTarget : MATLAB Function  TreatAsAtomicUnit=on
      settings: AttributesFormatString=实际状态到前轮角 / FrontAngleTarget
  LegacyAxleLoadMonitor : Terminator
      settings: AttributesFormatString=旧轴荷接口 / Legacy Loads
  LogActualLoadAllocation : ToWorkspace  VariableName=repair_actual_load_allocation  SaveFormat=Structure With Time  SampleTime=-1
      settings: AttributesFormatString=实际轮荷分配诊断 / Load Allocation
  Log_repair_wheel_diag : ToWorkspace  VariableName=repair_wheel_diag  SaveFormat=Timeseries  SampleTime=-1
      settings: AttributesFormatString=原始记录 repair_wheel_diag / Log_repair_wheel_diag
  LongitudinalForces : Mux  Inputs=2
      settings: AttributesFormatString=修正前后轴纵向力 / LongitudinalForces
  WheelTorqueBudget : MATLAB Function  TreatAsAtomicUnit=on
      settings: AttributesFormatString=实际轮荷分配与轮矩 / Actual Loads & Torque
  左前轮驱动力矩 : Outport
      settings: AttributesFormatString=左前轮驱动力矩 / Outport
  右前轮驱动力矩 : Outport  Port=2
      settings: AttributesFormatString=右前轮驱动力矩 / Outport
  左后轮驱动力矩 : Outport  Port=3
      settings: AttributesFormatString=左后轮驱动力矩 / Outport
  右后轮驱动力矩 : Outport  Port=4
      settings: AttributesFormatString=右后轮驱动力矩 / Outport
  FrontAngleCommand : Outport  Port=5
      settings: AttributesFormatString=前轮角目标 / FrontAngleCommand
  wires:
  左前轮实际轮速/1 -> ActualWheelSpeeds/1
  右前轮实际轮速/1 -> ActualWheelSpeeds/2
  左后轮实际轮速/1 -> ActualWheelSpeeds/3
  右后轮实际轮速/1 -> ActualWheelSpeeds/4
  前轴期望轴轮速/1 -> AxleSpeedTargets/1
  后轴期望轴轮速/1 -> AxleSpeedTargets/2
  前轴期望纵向力/1 -> LongitudinalForces/1
  后轴期望纵向力/1 -> LongitudinalForces/2
  前轴垂向力/1 -> ActualAxleLoads/1
  后轴垂向力/1 -> ActualAxleLoads/2
  V/1 -> ActualState/1
  beta/1 -> ActualState/2
  r/1 -> ActualState/3
  期望前轮侧偏角alpha_f_d/1 -> FrontAngleTarget/2(alpha)
  ActualState/1 -> WheelTorqueBudget/5(actual), FrontAngleTarget/1(actual)
  ActualWheelSpeeds/1 -> WheelTorqueBudget/1(omega)
  AxleSpeedTargets/1 -> WheelTorqueBudget/2(axis_w)
  FrontAngleTarget/1(delta) -> FrontAngleCommand/1
  LongitudinalForces/1 -> WheelTorqueBudget/3(Fx)
  WheelTorqueBudget/1(T_FL) -> 左前轮驱动力矩/1
  WheelTorqueBudget/2(T_FR) -> 右前轮驱动力矩/1
  WheelTorqueBudget/3(T_RL) -> 左后轮驱动力矩/1
  WheelTorqueBudget/4(T_RR) -> 右后轮驱动力矩/1
  WheelTorqueBudget/5(diag) -> Log_repair_wheel_diag/1
  [vec_WheelContact] -> WheelTorqueBudget/6(contact)
  MeasuredWheelContact/1 -> [vec_WheelContact]
  MeasuredFourWheelLoads/1 -> [measured_Fz4]
  [measured_Fz4] -> WheelTorqueBudget/4(Fz)
  ActualAxleLoads/1 -> LegacyAxleLoadMonitor/1
  WheelTorqueBudget/6(allocation_diag) -> LogActualLoadAllocation/1

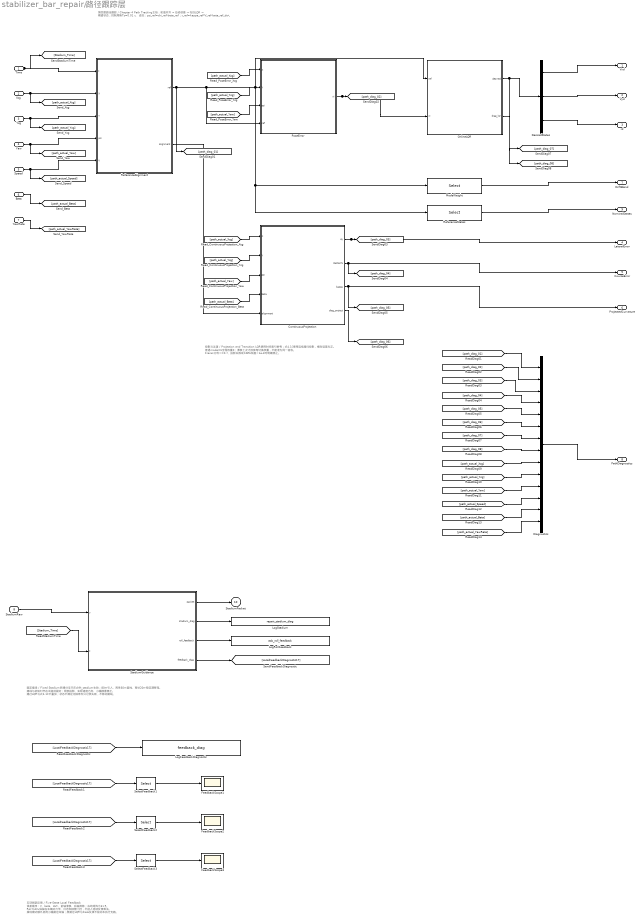
== system stabilizer_bar_repair/路径跟踪层 ==
  note: 第四章路径跟踪 / Chapter 4 Path Tracking
      | 主链：初值对齐 → 位姿误差 → 在线LQR → 期望状态；控制周期Ts=0.01 s。
      | 姿态：psi_ref=chi_ref-beta_ref；r_ref=kappa_ref*V_ref-beta_ref_dot。
  note: 投影与过渡 / Projection and Transition
      | LQR使用时间索引参考；式4.10使用连续路径投影，横向误差左正。
      | 普通mode=6全程权重0；漂移工况才按参考切换权重，不能混为同一验收。
      | Frenet分母<=0.1、投影失败或CARE残差>1e-8时明确停止。
  note: 固定操场 / Fixed Stadium
      | 新增分支只在drift_stadium生效；80m引入、两条60m直线、两处20m稳定漂移弯。
      | 路线与初始对齐在试验前固定；局部投影、实际速度方向、小幅横摆修正。
      | 路径LQR与式4.10不叠加；状态不满足切换条件只记录失败，不移动路线。
  note: 五项局部反馈 / Five-State Local Feedback
      | 误差顺序：V、beta、AVz、前轴滑移、后轴滑移；冻结矩阵为3×5。
      | Roll与AVx保留在车辆动力学、日志和接管门控，不进入连续反馈乘法。
      | 操场模式额外启用小幅路径纠偏；原路径LQR与Fiala反演不驱动本执行支路。
  Time : Inport
      settings: AttributesFormatString=采样时刻 / Time
  Xcg : Inport  Port=2
      settings: AttributesFormatString=实际质心X / Xcg
  Ycg : Inport  Port=3
      settings: AttributesFormatString=实际质心Y / Ycg
  Yaw : Inport  Port=4
      settings: AttributesFormatString=实际航向角 / Yaw
  Speed : Inport  Port=5
      settings: AttributesFormatString=实际总车速 / Speed
  Beta : Inport  Port=6
      settings: AttributesFormatString=实际侧偏角 / Beta
  YawRate : Inport  Port=7
      settings: AttributesFormatString=实际横摆角速度 / YawRate
  StadiumRaw : Inport  Port=8
      settings: AttributesFormatString=操场实测原始状态 / Stadium Raw State
  ContinuousProjection : MATLAB Function  TreatAsAtomicUnit=on
      settings: AttributesFormatString=连续路径投影 / ContinuousProjection
  DesiredStates : Demux  Outputs=3
      settings: AttributesFormatString=期望状态分解 / DesiredStates
  Diagnostics : Mux  Inputs=14
      settings: AttributesFormatString=原始诊断汇总 / Diagnostics
  FeedbackScope1 : Scope
      settings: AttributesFormatString=直接侧倾反馈为零 / Zero Direct Roll Feedback
  FeedbackScope2 : Scope
      settings: AttributesFormatString=名义前馈与实际请求 / Feedforward and Request
  FeedbackScope3 : Scope
      settings: AttributesFormatString=阶段失败原因 / Stage Failure Causes
  LogFeedbackDiagnostic : ToWorkspace  VariableName=feedback_diag  SaveFormat=Structure With Time  SampleTime=-1
      settings: AttributesFormatString=五项反馈诊断 / Five-State Feedback Diagnostic
  LogRollFeedback : ToWorkspace  VariableName=asb_roll_feedback  SaveFormat=Structure With Time  SampleTime=-1
      settings: AttributesFormatString=记录两项零贡献 / Log Zero Roll Contributions
  LogStadium : ToWorkspace  VariableName=repair_stadium_diag  SaveFormat=Structure With Time  SampleTime=-1
      settings: AttributesFormatString=操场进度误差与失败记录 / Stadium Diagnostics
  ModeWeight : Selector  InputPortWidth=14  IndexOptions=Index vector (dialog)  Indices=10  OutputSizes=1
      settings: AttributesFormatString=平滑漂移权重 / ModeWeight
  OnlineLQR : MATLAB Function  TreatAsAtomicUnit=on
      settings: AttributesFormatString=在线连续LQR / OnlineLQR
  PoseError : MATLAB Function  TreatAsAtomicUnit=on
      settings: AttributesFormatString=全局位姿误差 / PoseError
  ReferenceAlignment : MATLAB Function  Description=|  TreatAsAtomicUnit=on
      | 默认mode=6普通轨迹：40m直线→25m入弯→40m定曲率→25m出弯→直线。
      | R=80m，V=10.5m/s，beta_ref=0，drift_blend=0。
      | 阶段1至5分别记录；不与入漂、退漂试验混淆。
      settings: AttributesFormatString=参考工况与初值对齐 / Reference Alignment
  ReferenceStates : Selector  InputPortWidth=14  IndexOptions=Index vector (dialog)  Indices=[7 8 6]  OutputSizes=1
      settings: AttributesFormatString=名义参考状态 / ReferenceStates
  SelectFeedback1 : Selector  InputPortWidth=17  IndexOptions=Index vector (dialog)  Indices=[2:7]  OutputSizes=1
      settings: AttributesFormatString=选择诊断项 / Select Diagnostic
  SelectFeedback2 : Selector  InputPortWidth=17  IndexOptions=Index vector (dialog)  Indices=[8:13]  OutputSizes=1
      settings: AttributesFormatString=选择诊断项 / Select Diagnostic
  SelectFeedback3 : Selector  InputPortWidth=17  IndexOptions=Index vector (dialog)  Indices=[14:17]  OutputSizes=1
      settings: AttributesFormatString=选择诊断项 / Select Diagnostic
  StadiumGuidance : MATLAB Function  TreatAsAtomicUnit=on
      settings: AttributesFormatString=五项反馈与路径纠偏 / Five-State Guidance
  Vxd : Outport
      settings: AttributesFormatString=期望纵向速度 / Vxd
  Vyd : Outport  Port=2
      settings: AttributesFormatString=期望侧向速度 / Vyd
  rd : Outport  Port=3
      settings: AttributesFormatString=期望横摆角速度 / rd
  LateralError : Outport  Port=4
      settings: AttributesFormatString=左正横向误差 / LateralError
  CourseError : Outport  Port=5
      settings: AttributesFormatString=速度方向误差 / CourseError
  ProjectedCurvature : Outport  Port=6
      settings: AttributesFormatString=投影路径曲率 / ProjectedCurvature
  DriftBlend : Outport  Port=7
      settings: AttributesFormatString=漂移模式权重 / DriftBlend
  PathDiagnostics : Outport  Port=8
      settings: AttributesFormatString=路径诊断 / PathDiagnostics
  NominalStates : Outport  Port=9
      settings: AttributesFormatString=名义参考V_beta_r / NominalStates
  StadiumPacket : Outport  Port=10
      settings: AttributesFormatString=操场唯一执行参考 / Stadium Packet
  wires:
  Xcg/1 -> [path_actual_Xcg], ReferenceAlignment/2(X)
  Ycg/1 -> [path_actual_Ycg], ReferenceAlignment/3(Y)
  Yaw/1 -> [path_actual_Yaw], ReferenceAlignment/4(psi)
  Speed/1 -> [path_actual_Speed], ReferenceAlignment/5(V)
  Beta/1 -> [path_actual_Beta]
  YawRate/1 -> [path_actual_YawRate]
  Time/1 -> ReferenceAlignment/1(t), [Stadium_Time]
  [path_actual_Xcg] -> PoseError/1(X)
  [path_actual_Ycg] -> PoseError/2(Y)
  [path_actual_Yaw] -> PoseError/3(psi)
  ReferenceAlignment/1(ref) -> ModeWeight/1, ReferenceStates/1, OnlineLQR/1(ref), PoseError/4(ref), [path_diag_01]
  PoseError/1(xi) -> OnlineLQR/2(xi), [path_diag_02]
  OnlineLQR/1(desired) -> DesiredStates/1, [path_diag_08]
  [path_actual_Xcg] -> ContinuousProjection/1(X)
  [path_actual_Ycg] -> ContinuousProjection/2(Y)
  [path_actual_Yaw] -> ContinuousProjection/3(psi)
  [path_actual_Beta] -> ContinuousProjection/4(beta)
  ReferenceAlignment/2(alignment) -> ContinuousProjection/5(alignment)
  DesiredStates/1 -> Vxd/1
  DesiredStates/2 -> Vyd/1
  DesiredStates/3 -> rd/1
  ContinuousProjection/1(ey) -> LateralError/1, [path_diag_03]
  ContinuousProjection/2(DeltaChi) -> CourseError/1, [path_diag_04]
  ContinuousProjection/3(kappa) -> ProjectedCurvature/1, [path_diag_05]
  ModeWeight/1 -> DriftBlend/1
  Diagnostics/1 -> PathDiagnostics/1
  ReferenceStates/1 -> NominalStates/1
  [path_diag_01] -> Diagnostics/1
  [path_diag_02] -> Diagnostics/2
  [path_diag_03] -> Diagnostics/3
  [path_diag_04] -> Diagnostics/4
  [path_diag_05] -> Diagnostics/5
  ContinuousProjection/4(diag_project) -> [path_diag_06]
  [path_diag_06] -> Diagnostics/6
  OnlineLQR/2(diag_lqr) -> [path_diag_07]
  [path_diag_07] -> Diagnostics/7
  [path_diag_08] -> Diagnostics/8
  [path_actual_Xcg] -> Diagnostics/9
  [path_actual_Ycg] -> Diagnostics/10
  [path_actual_Yaw] -> Diagnostics/11
  [path_actual_Speed] -> Diagnostics/12
  [path_actual_Beta] -> Diagnostics/13
  [path_actual_YawRate] -> Diagnostics/14
  StadiumRaw/1 -> StadiumGuidance/1(y)
  [Stadium_Time] -> StadiumGuidance/2(t)
  [LocalFeedbackDiagnostic17] -> LogFeedbackDiagnostic/1
  [LocalFeedbackDiagnostic17] -> SelectFeedback1/1
  SelectFeedback1/1 -> FeedbackScope1/1
  [LocalFeedbackDiagnostic17] -> SelectFeedback2/1
  SelectFeedback2/1 -> FeedbackScope2/1
  [LocalFeedbackDiagnostic17] -> SelectFeedback3/1
  SelectFeedback3/1 -> FeedbackScope3/1
  StadiumGuidance/1(packet) -> StadiumPacket/1
  StadiumGuidance/2(stadium_diag) -> LogStadium/1
  StadiumGuidance/3(roll_feedback) -> LogRollFeedback/1
  StadiumGuidance/4(feedback_diag) -> [LocalFeedbackDiagnostic17]

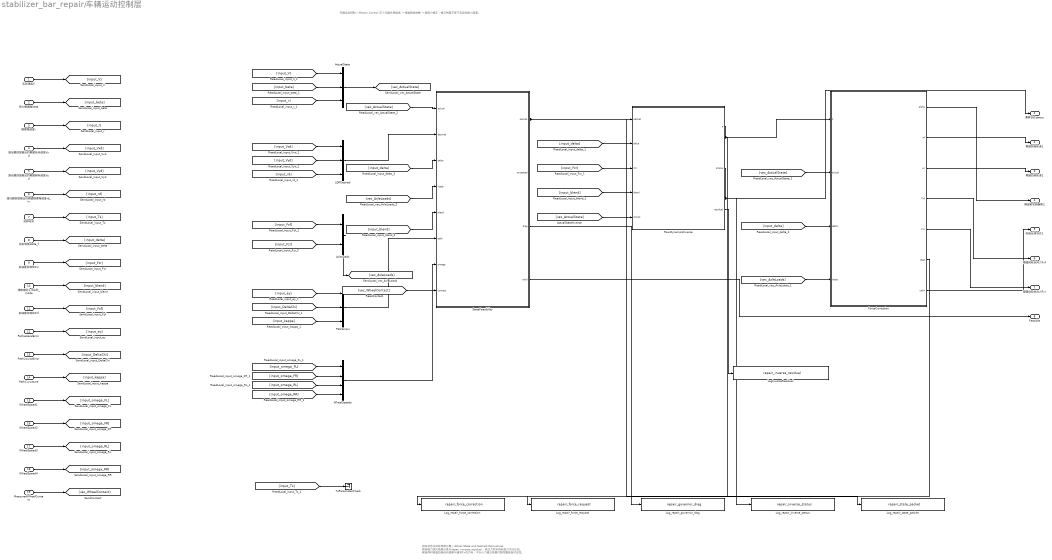
== system stabilizer_bar_repair/车辆运动控制层 ==
  note: 车辆运动控制 / Motion Control
      | 33个无副作用候选 → 保留原始逆解 → 局部力修正；修正残差不等于实际轮胎力误差。
  note: 实际状态与目标导数分离 / Actual State and Desired Derivatives
      | 原始轴力回代残差记录为repair_inverse_residual；修正力和实际轮胎力另行比较。
      | 候选同时检查后轴纵向滑移与请求Fx的方向；不以小力修正残差代替完整轮胎可达性。
  实际速度V : Inport
      settings: AttributesFormatString=总速度 / V
  质心侧偏角beta : Inport  Port=2
      settings: AttributesFormatString=质心侧偏角 / beta
  横摆角速度r : Inport  Port=3
      settings: AttributesFormatString=横摆角速度 / r
  路径跟踪层输出的期望纵向速度Vxd : Inport  Port=4
      settings: AttributesFormatString=LQR纵向目标 / Vxd
  路径跟踪层输出的期望侧向速度Vyd : Inport  Port=5
      settings: AttributesFormatString=LQR侧向目标 / Vyd
  路径跟踪层输出的期望横摆角速度rd_in : Inport  Port=6
      settings: AttributesFormatString=LQR横摆目标 / rd
  采样时间 : Inport  Port=7
      settings: AttributesFormatString=控制周期 / Ts
  前轮转角delta_f : Inport  Port=8
      settings: AttributesFormatString=实测前轮角 / delta
  后轴垂向载荷Fzr : Inport  Port=9
      settings: AttributesFormatString=实测后轴载荷 / Fzr
  漂移模式1_0drift_mode : Inport  Port=10
      settings: AttributesFormatString=漂移权重 / blend
  前轴垂向载荷Fzf : Inport  Port=11
      settings: AttributesFormatString=实测前轴载荷 / Fzf
  PathLateralError : Inport  Port=12
      settings: AttributesFormatString=左正横向误差 / ey
  PathCourseError : Inport  Port=13
      settings: AttributesFormatString=速度方向误差 / DeltaChi
  PathCurvature : Inport  Port=14
      settings: AttributesFormatString=投影曲率 / kappa
  WheelSpeed1 : Inport  Port=15
      settings: AttributesFormatString=左前实际轮速 / omega_FL
  WheelSpeed2 : Inport  Port=16
      settings: AttributesFormatString=右前实际轮速 / omega_FR
  WheelSpeed3 : Inport  Port=17
      settings: AttributesFormatString=左后实际轮速 / omega_RL
  WheelSpeed4 : Inport  Port=18
      settings: AttributesFormatString=右后实际轮速 / omega_RR
  MeasuredWheelContact : Inport  Port=19
      settings: AttributesFormatString=实测轮胎负载 / Contact
  ActualState : Mux  Inputs=3
      settings: AttributesFormatString=实际V beta r / ActualState
  AxleLoads : Mux  Inputs=2
      settings: AttributesFormatString=实际前后轴载荷 / AxleLoads
  ForceCorrection : MATLAB Function  TreatAsAtomicUnit=on
      settings: AttributesFormatString=连续力修正与轮速反演 / ForceCorrection
  LQRDesired : Mux  Inputs=3
      settings: AttributesFormatString=LQR原始期望 / LQRDesired
  LogInverseResidual : ToWorkspace  VariableName=repair_inverse_residual  SaveFormat=Timeseries  SampleTime=-1
      settings: AttributesFormatString=实际状态回代残差 / Inverse Residual
  Log_repair_force_correction : ToWorkspace  VariableName=repair_force_correction  SaveFormat=Timeseries  SampleTime=-1
      settings: AttributesFormatString=原始记录 repair_force_correction / Log_repair_force_correction
  Log_repair_force_request : ToWorkspace  VariableName=repair_force_request  SaveFormat=Timeseries  SampleTime=-1
      settings: AttributesFormatString=原始记录 repair_force_request / Log_repair_force_request
  Log_repair_governor_diag : ToWorkspace  VariableName=repair_governor_diag  SaveFormat=Timeseries  SampleTime=-1
      settings: AttributesFormatString=原始记录 repair_governor_diag / Log_repair_governor_diag
  Log_repair_inverse_status : ToWorkspace  VariableName=repair_inverse_status  SaveFormat=Timeseries  SampleTime=-1
      settings: AttributesFormatString=原始记录 repair_inverse_status / Log_repair_inverse_status
  Log_repair_state_packet : ToWorkspace  VariableName=repair_state_packet  SaveFormat=Timeseries  SampleTime=-1
      settings: AttributesFormatString=原始记录 repair_state_packet / Log_repair_state_packet
  PathErrors : Mux  Inputs=3
      settings: AttributesFormatString=路径误差与曲率 / PathErrors
  RawDynamicsInverse : MATLAB Function  TreatAsAtomicUnit=on
      settings: AttributesFormatString=实际状态动力学逆解 / Actual-state Inverse
  StateFeasibility : MATLAB Function  TreatAsAtomicUnit=on
      settings: AttributesFormatString=状态误差与候选可行性 / StateFeasibility
  TsParameterCheck : Terminator
      settings: AttributesFormatString=采样数值仅作兼容 / TsParameterCheck
  WheelSpeeds : Mux
      settings: AttributesFormatString=四轮实际角速度 / WheelSpeeds
  漂移状态status : Outport
      settings: AttributesFormatString=原逆解状态 / inverse_status
  期望前轴轮速1 : Outport  Port=2
      settings: AttributesFormatString=前轴候选轮速 / omega_f
  期望后轴轮速1 : Outport  Port=3
      settings: AttributesFormatString=后轴候选轮速 / omega_r
  期望前轮侧偏角2 : Outport  Port=4
      settings: AttributesFormatString=前轴目标侧偏角 / alpha_f
  轮胎反演状态1 : Outport  Port=5
      settings: AttributesFormatString=反演有效标志 / force_valid
  期望前轮纵向力Fxf : Outport  Port=6
      settings: AttributesFormatString=修正前轴纵向力 / Fxf
  期望后轮纵向力Fxr : Outport  Port=7
      settings: AttributesFormatString=修正后轴纵向力 / Fxr
  Feasible : Outport  Port=8
      settings: AttributesFormatString=候选可行标志 / candidate_valid
  wires:
  实际速度V/1 -> [input_V]
  质心侧偏角beta/1 -> [input_beta]
  横摆角速度r/1 -> [input_r]
  路径跟踪层输出的期望纵向速度Vxd/1 -> [input_Vxd]
  路径跟踪层输出的期望侧向速度Vyd/1 -> [input_Vyd]
  路径跟踪层输出的期望横摆角速度rd_in/1 -> [input_rd]
  采样时间/1 -> [input_Ts]
  前轮转角delta_f/1 -> [input_delta]
  后轴垂向载荷Fzr/1 -> [input_Fzr]
  漂移模式1_0drift_mode/1 -> [input_blend]
  前轴垂向载荷Fzf/1 -> [input_Fzf]
  PathLateralError/1 -> [input_ey]
  PathCourseError/1 -> [input_DeltaChi]
  PathCurvature/1 -> [input_kappa]
  WheelSpeed1/1 -> [input_omega_FL]
  WheelSpeed2/1 -> [input_omega_FR]
  WheelSpeed3/1 -> [input_omega_RL]
  WheelSpeed4/1 -> [input_omega_RR]
  ActualState/1 -> [vec_ActualState]
  AxleLoads/1 -> [vec_AxleLoads]
  ForceCorrection/1(alpha) -> 期望前轮侧偏角2/1
  ForceCorrection/2(wf) -> 期望前轴轮速1/1
  ForceCorrection/3(wr) -> 期望后轴轮速1/1
  ForceCorrection/4(Fxf) -> 期望前轮纵向力Fxf/1
  ForceCorrection/5(Fxr) -> 期望后轮纵向力Fxr/1
  ForceCorrection/6(diag) -> Log_repair_force_correction/1
  ForceCorrection/7(valid) -> 轮胎反演状态1/1
  LQRDesired/1 -> StateFeasibility/2(desired)
  PathErrors/1 -> StateFeasibility/6(path)
  RawDynamicsInverse/1(F) -> ForceCorrection/1(F), Log_repair_force_request/1
  RawDynamicsInverse/2(status) -> 漂移状态status/1, Log_repair_inverse_status/1
  [input_DeltaChi] -> PathErrors/2
  [input_Fzf] -> AxleLoads/1
  [input_Fzr] -> AxleLoads/2
  [input_Ts] -> TsParameterCheck/1
  [input_V] -> ActualState/1
  [input_Vxd] -> LQRDesired/1
  [input_Vyd] -> LQRDesired/2
  [input_beta] -> ActualState/2
  [input_blend] -> StateFeasibility/5(blend)
  [input_delta] -> ForceCorrection/3(delta)
  [input_delta] -> StateFeasibility/3(delta)
  [input_ey] -> PathErrors/1
  [input_kappa] -> PathErrors/3
  [input_omega_FL] -> WheelSpeeds/1
  [input_omega_FR] -> WheelSpeeds/2
  [input_omega_RL] -> WheelSpeeds/3
  [input_omega_RR] -> WheelSpeeds/4
  [input_r] -> ActualState/3
  [input_rd] -> LQRDesired/3
  [vec_ActualState] -> ForceCorrection/2(actual)
  [vec_ActualState] -> StateFeasibility/1(actual)
  [vec_AxleLoads] -> ForceCorrection/4(loads)
  [vec_AxleLoads] -> StateFeasibility/4(loads)
  StateFeasibility/1(packet) -> RawDynamicsInverse/1(packet), Log_repair_state_packet/1
  StateFeasibility/3(diag) -> Log_repair_governor_diag/1
  StateFeasibility/4(valid) -> Feasible/1
  WheelSpeeds/1 -> StateFeasibility/7(omega)
  [vec_ActualState] -> RawDynamicsInverse/5(actual)
  [input_delta] -> RawDynamicsInverse/2(delta)
  [input_Fzr] -> RawDynamicsInverse/3(Fzr)
  [input_blend] -> RawDynamicsInverse/4(blend)
  RawDynamicsInverse/3(residual) -> LogInverseResidual/1
  [vec_WheelContact] -> StateFeasibility/8(contact)
  MeasuredWheelContact/1 -> [vec_WheelContact]

== matlab function stabilizer_bar_repair/执行器调节层/WheelTorqueBudget ==
  settings: updateMethod=DISCRETE  sampleTime=Ts
  data: omega input size=[4 1]; T_FL output; axis_w input size=[2 1]; Fx input size=[2 1]; Fz input size=[4 1]; actual input size=[3 1]; contact input size=[8 1]; T_FR output; T_RL output; T_RR output; diag output size=[71 1]; repair_cfg parameter; allocation_diag output size=[28 1]
function [T_FL,T_FR,T_RL,T_RR,diag,allocation_diag] = wheel_execution(omega,axis_w,Fx,Fz,actual,contact,repair_cfg)
%#codegen
% 使用CarSim实际四轮轮荷分配轴级纵向力，保留原正式模式的轮速控制律。
% Fz和omega轮序为FL/FR/RL/RR，单位N和rad/s；Fx为前后轴目标纵向力N。
% contact前四项为实际轮胎纵向力N。本修改不改变悬架、轮胎表或原控制增益。
% allocation_diag记录真实轮荷、权重、目标/实际轮力、未实现轴力和附加横摆力矩。
persistent previous initialized
if isempty(initialized),previous=zeros(4,1);initialized=false;end
assert(all(isfinite(Fz)),'Nonfinite measured normal loads'); % 非有限轮荷无法参与物理分配。
Fxd=zeros(4,1);weights=zeros(4,1);unserved=zeros(2,1);lost=Fz<=0;
for ax=1:2
    i=2*ax-1;j=2*ax;
    % 非接地轮不承接分配力；max仅用于权重，原负轮荷和失载标志保留。
    l=max(Fz(i),0);r=max(Fz(j),0);total=l+r;
    if total>1
        weights(i)=l/total;weights(j)=r/total;
        Fxd(i)=weights(i)*Fx(ax);Fxd(j)=Fx(ax)-Fxd(i);
    else
        unserved(ax)=Fx(ax); % 整轴失载：不静默假定存在可实现的纵向力。
    end
end
V=actual(1);beta=actual(2);r=actual(3);ay=V*r*cos(beta);
offset=repair_cfg.d*r/(2*repair_cfg.Rw);
wd=[axis_w(1)-offset;axis_w(1)+offset;axis_w(2)-offset;axis_w(2)+offset];
if initialized,dwd=(wd-previous)/repair_cfg.Ts;else,dwd=zeros(4,1);end
omega=omega(1:4);feedback=repair_cfg.kw*(wd-omega);inertia=repair_cfg.Iw*dwd;
loadTorque=repair_cfg.Rw*Fxd;raw=feedback+inertia+loadTorque;T=raw;
rearSlipPower=Fx(2)*(repair_cfg.Rw*axis_w(2)-V*cos(beta));
% 旧日志通道顺序保持不变，新增分配日志另走独立输出。
diag=[raw;T;wd;omega;zeros(4,1);dwd;Fxd;ay;wd;zeros(4,1); ...
 feedback;inertia;loadTorque;zeros(4,1);repair_cfg.kw*ones(4,1); ...
 zeros(2,1);zeros(2,1);contact(1:4);contact(1:4)-Fxd;rearSlipPower;1];
frontDiff=Fz(2)-Fz(1);rearDiff=Fz(4)-Fz(3);totalDiff=frontDiff+rearDiff;
ratioValid=abs(totalDiff)>=100;pf=NaN;pr=NaN;
if ratioValid,pf=frontDiff/totalDiff;pr=rearDiff/totalDiff;end
% 这里仅记录纵向轮力差产生的横摆力矩（未旋转到实际前轮角）；
% 完整车体合力和力矩残差在原始轮力、转角和轴力日志中离线计算。
MzLong=repair_cfg.d/2*(Fxd(2)-Fxd(1)+Fxd(4)-Fxd(3));
allocation_diag=[Fz(:);weights;Fx(:);Fxd;contact(1:4);unserved; ...
 double(lost(:));pf;pr;double(ratioValid);MzLong];
previous=wd;initialized=true;T_FL=T(1);T_FR=T(2);T_RL=T(3);T_RR=T(4);
end

== matlab function stabilizer_bar_repair/执行器调节层/FrontAngleTarget ==
  settings: updateMethod=DISCRETE  sampleTime=Ts
  data: actual input size=[3 1]; delta output; alpha input; repair_cfg parameter
function delta=front_target(actual,alpha,repair_cfg)
% 实际V/beta/r推导前轴接地点方向，单位rad。
delta=atan2(actual(1)*sin(actual(2))+repair_cfg.a*actual(3),actual(1)*cos(actual(2)))-alpha;
end
